simulink subsystem "Subsys_Conv_Electrical_Part_SPS"  (R2022b)
settings: Solver=VariableStepAuto  StartTime=0.0  StopTime=10.0  RelTol=1e-3
model mask{S_n=2e6, f_n=50, V_n_phph=690, V_n_grid_phph=20e3, T_s_ctrl=1e-3, T_s_meas=1e-4, T_s_SPS=1e-4, datatype='double', L_filter_conv_pu=[ 0.005 0.23 ], C_filter_pu=[ 0.005 0.01 ], L_filter_grid_pu=[ 0.01 0.04 ], withTransformer=1, RL_Trafo_Conv=[ 0.005 0.02 ], RL_Trafo_Grid=[ 0.005 0.02 ], Rm=500, Lm=500, inverterModel=1, R_snubber_pu=5e6, R_on_pu=1e-3, energySourceModel=1, C_dc_pu=0.75, K_p_DC=1.2, K_i_DC=2.4}
  mask prompts: S_n "Nominal Apparent Power [VA]"; f_n "Nominal Frequency [Hz]"; V_n_phph "Nominal Converter Voltage (rms, ph-ph) [V]"; V_n_grid_phph "Nominal Grid Voltage (rms, ph-ph) [V]"; T_s_ctrl "DC-link voltage controller sample time [s]"; T_s_meas "Measurement sample time [s]"; T_s_SPS "Simscape SPS sample time [s]"; datatype "Measurement signal data type"; L_filter_conv_pu "Impedance of Converter-Side-Inductor [ R L ] (p.u.)"; C_filter_pu "Impedance of Filter Capacitor [ R C ] (p.u.)"; L_filter_grid_pu "Impedance of Grid-Side-Inductor (only if no transformer used) [ R L ] (p.u.)"; withTransformer "Grid coupling: (1 = with transformer, 0 = direct grid coupling (without transformer)"; RL_Trafo_Conv "Converter-Side Impedance [ R L ] (pu):"; RL_Trafo_Grid "Grid-Side Impedance [ R L ] (pu):"; Rm "Magnetization resistance  Rm (pu):"; Lm "Magnetization inductance  Lm (pu):"; inverterModel "Modeling of inverter brigde: (1 = Average Model, 0 = Ideal Switches)"; R_snubber_pu "Snubber Resistance for Ideal Switches (pu)"; R_on_pu "On-State Resistance of Ideal Switches (pu)"; energySourceModel "Modeling of energy source (1 = power-limited DC current source , 0 = constant DC voltage)"; C_dc_pu "Capacitance of DC-link capacitor (pu)"; K_p_DC "Current controller proportional gain (pu)"; K_i_DC "Current controller integral gain (pu/s)"
undefined symbols (not defined in the file): D1, Delta
libraries: spsThreePhaseVIMeasurementLib x6, spsIdealSwitchLib x3, spsThreePhaseSeriesRLCBranchLib x3, spsUniversalBridgeLib x2, spsVoltageMeasurementLib x2, spsGroundLib x1, spsDCVoltageSourceLib x1, spsControlledCurrentSourceLib x1, slpidlib x1, spsSeriesRLCBranchLib x1, spsThreePhaseBreakerLib x1, spsThreePhaseTransformerTwoWindingsLib x1
settings Model: Creator=winkens  LastModifiedBy=winkens
settings SolverCC: AlgebraicLoopSolver=TrustRegion
settings DebuggingCC: UnconnectedInputMsg=warning  UnconnectedOutputMsg=warning  UnconnectedLineMsg=warning  SFMachineParentedDataDiag=warning
settings ModelReferenceCC: EnableRefExpFcnMdlSchedulingChecks=on
settings RTWCC: DLArmComputeVersion=19.05

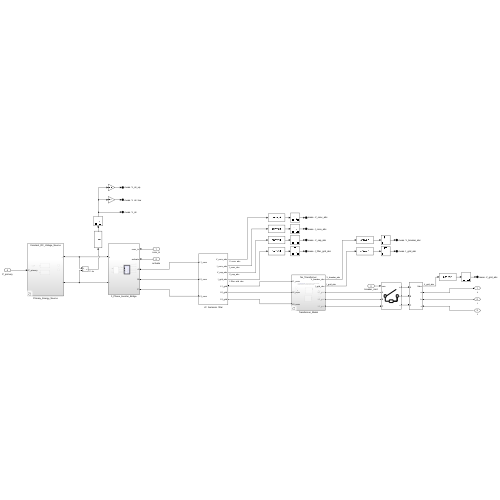
[thumbnail: Simulink's stored preview of the top-level diagram]
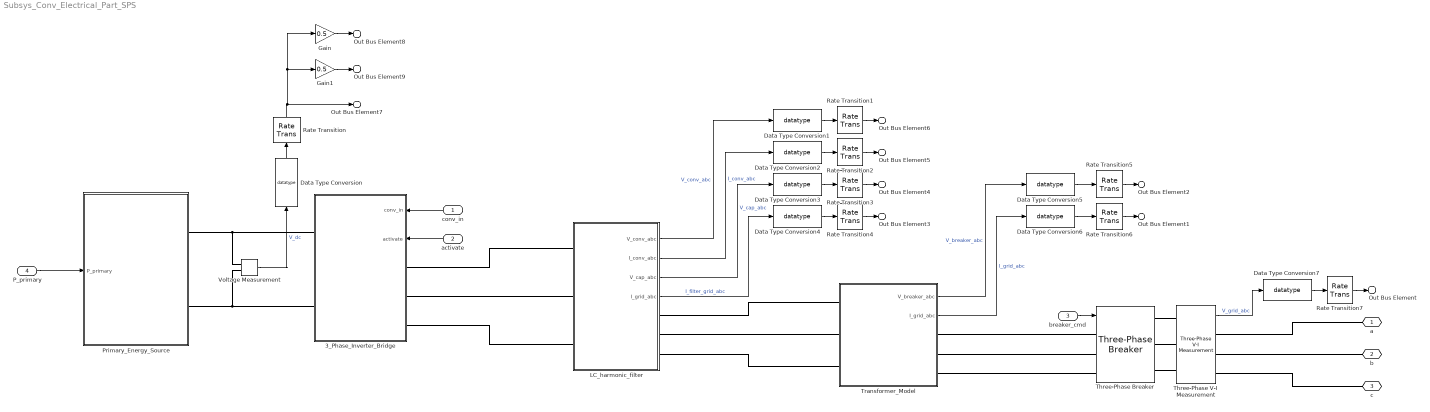
== system Subsys_Conv_Electrical_Part_SPS ==
  conv_in : Inport
  activate : Inport  Port=2
  breaker_cmd : Inport  Port=3
  P_primary : Inport  Port=4
  3_Phase_Inverter_Bridge : Subsystem
  Data Type Conversion{,1..7} (8 alike) : DataTypeConversion  OutDataTypeStr=datatype  SaturateOnIntegerOverflow=off  RndMeth=Floor
  Gain : Gain  Gain=0.5
  Gain1 : Gain  Gain=0.5
  LC_harmonic_filter : Subsystem
  Primary_Energy_Source : Subsystem  Variant=on
  Rate Transition{,1..7} (8 alike) : RateTransition  OutPortSampleTime=T_s_meas
  Three-Phase V-I Measurement : spsThreePhaseVIMeasurementLib/Three-Phase V-I Measurement  VoltageMeasurement=phase-to-ground  SetLabelV=off  LabelV=Vabc  Vpu=off  VpuLL=off  CurrentMeasurement=no  SetLabelI=off  LabelI=Iabc  Ipu=off  Pbase=100e6  Vbase=500e3  OutputType=Complex  PhasorSimulation=off  PSBequivalent=0
  Three-Phase Breaker : spsThreePhaseBreakerLib/Three-Phase Breaker  InitialState=open  SwitchA=on  SwitchB=on  SwitchC=on  SwitchTimes="[1/60  5/60]"  External=on  BreakerResistance=0.01  SnubberResistance=1e6  SnubberCapacitance=inf  Measurements=None
  Transformer_Model : Subsystem  Variant=on
  Voltage Measurement : spsVoltageMeasurementLib/Voltage Measurement  PhasorSimulation=off  OutputType=Complex  PSBequivalent=0
  a : PMIOPort  Side=Right
  b : PMIOPort  Port=2  Side=Right
  c : PMIOPort  Port=3  Side=Right
  Out Bus Element : Outport  PortName=meas  Element=V_grid_abc
  Out Bus Element1 : Outport  PortName=meas  Element=I_grid_abc
  Out Bus Element2 : Outport  PortName=meas  Element=V_breaker_abc
  Out Bus Element3 : Outport  PortName=meas  Element=I_filter_grid_abc
  Out Bus Element4 : Outport  PortName=meas  Element=V_cap_abc
  Out Bus Element5 : Outport  PortName=meas  Element=I_conv_abc
  Out Bus Element6 : Outport  PortName=meas  Element=V_conv_abc
  Out Bus Element7 : Outport  PortName=meas  Element=V_dc
  Out Bus Element8 : Outport  PortName=meas  Element=V_dc_up
  Out Bus Element9 : Outport  PortName=meas  Element=V_dc_low
  wires:
  LC_harmonic_filter/4(I_grid_abc) -> Data Type Conversion4/1  "I_filter_grid_abc"
  breaker_cmd/1 -> Three-Phase Breaker/1
  Transformer_Model/1(V_breaker_abc) -> Data Type Conversion5/1  "V_breaker_abc"
  LC_harmonic_filter/2(I_conv_abc) -> Data Type Conversion2/1  "I_conv_abc"
  LC_harmonic_filter/3(V_cap_abc) -> Data Type Conversion3/1  "V_cap_abc"
  Voltage Measurement/1 -> Data Type Conversion/1  "V_dc"
  Three-Phase V-I Measurement/1 -> Data Type Conversion7/1  "V_grid_abc"
  LC_harmonic_filter/1(V_conv_abc) -> Data Type Conversion1/1  "V_conv_abc"
  Transformer_Model/2(I_grid_abc) -> Data Type Conversion6/1  "I_grid_abc"
  P_primary/1 -> Primary_Energy_Source/1(P_primary)
  activate/1 -> 3_Phase_Inverter_Bridge/2(activate)
  conv_in/1 -> 3_Phase_Inverter_Bridge/1(conv_in)
  Gain/1 -> Out Bus Element8/1
  Gain1/1 -> Out Bus Element9/1
  Rate Transition/1 -> Out Bus Element7/1, Gain/1, Gain1/1
  Rate Transition1/1 -> Out Bus Element6/1
  Rate Transition2/1 -> Out Bus Element5/1
  Rate Transition3/1 -> Out Bus Element4/1
  Rate Transition4/1 -> Out Bus Element3/1
  Rate Transition5/1 -> Out Bus Element2/1
  Rate Transition6/1 -> Out Bus Element1/1
  Rate Transition7/1 -> Out Bus Element/1
  Data Type Conversion/1 -> Rate Transition/1
  Data Type Conversion1/1 -> Rate Transition1/1
  Data Type Conversion2/1 -> Rate Transition2/1
  Data Type Conversion3/1 -> Rate Transition3/1
  Data Type Conversion4/1 -> Rate Transition4/1
  Data Type Conversion5/1 -> Rate Transition5/1
  Data Type Conversion6/1 -> Rate Transition6/1
  Data Type Conversion7/1 -> Rate Transition7/1
  connections:
  Voltage Measurement/LConn1 -- Primary_Energy_Source/RConn1 -- 3_Phase_Inverter_Bridge/RConn1
  Primary_Energy_Source/RConn2 -- Voltage Measurement/LConn2 -- 3_Phase_Inverter_Bridge/RConn2
  Three-Phase V-I Measurement/RConn2 -- b/RConn1
  Three-Phase V-I Measurement/RConn1 -- a/RConn1
  LC_harmonic_filter/LConn3 -- 3_Phase_Inverter_Bridge/LConn3
  Three-Phase Breaker/LConn3 -- Transformer_Model/RConn3
  Three-Phase V-I Measurement/LConn2 -- Three-Phase Breaker/RConn2
  Three-Phase V-I Measurement/RConn3 -- c/RConn1
  Three-Phase V-I Measurement/LConn1 -- Three-Phase Breaker/RConn1
  Three-Phase V-I Measurement/LConn3 -- Three-Phase Breaker/RConn3
  Three-Phase Breaker/LConn1 -- Transformer_Model/RConn1
  LC_harmonic_filter/RConn1 -- Transformer_Model/LConn1
  Three-Phase Breaker/LConn2 -- Transformer_Model/RConn2
  LC_harmonic_filter/RConn3 -- Transformer_Model/LConn3
  Transformer_Model/LConn2 -- LC_harmonic_filter/RConn2
  LC_harmonic_filter/LConn1 -- 3_Phase_Inverter_Bridge/LConn1
  LC_harmonic_filter/LConn2 -- 3_Phase_Inverter_Bridge/LConn2

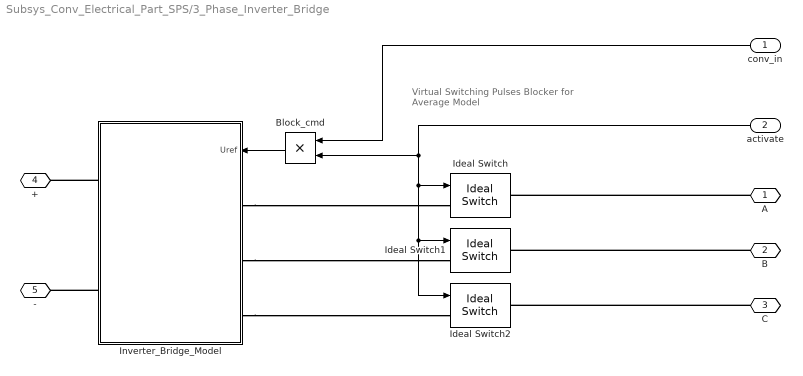
== system Subsys_Conv_Electrical_Part_SPS/3_Phase_Inverter_Bridge ==
  note: Virtual Switching Pulses
      | Blocker for Average Model
  conv_in : Inport
  activate : Inport  Port=2
  Block_cmd : Product  Inputs=**
  Ideal Switch : spsIdealSwitchLib/Ideal Switch  Ron=1e-6 * V_n_phph * V_n_phph / S_n  Lon=0  IC=1  Rs=1e6 * V_n_phph * V_n_phph / S_n  Cs=inf  Measurements=off
  Ideal Switch1 : spsIdealSwitchLib/Ideal Switch  Ron=1e-6 * V_n_phph * V_n_phph / S_n  Lon=0  IC=1  Rs=1e6 * V_n_phph * V_n_phph / S_n  Cs=inf  Measurements=off
  Ideal Switch2 : spsIdealSwitchLib/Ideal Switch  Ron=1e-6 * V_n_phph * V_n_phph / S_n  Lon=0  IC=1  Rs=1e6 * V_n_phph * V_n_phph / S_n  Cs=inf  Measurements=off
  Inverter_Bridge_Model : Subsystem  Variant=on  VariantControl=Choice
  A : PMIOPort  Side=Left
  B : PMIOPort  Port=2  Side=Left
  C : PMIOPort  Port=3  Side=Left
  + : PMIOPort  Port=4  Side=Right
  - : PMIOPort  Port=5  Side=Right
  wires:
  conv_in/1 -> Block_cmd/1
  activate/1 -> Ideal Switch/1, Ideal Switch1/1, Ideal Switch2/1, Block_cmd/2
  Block_cmd/1 -> Inverter_Bridge_Model/1(Uref)
  connections:
  C/RConn1 -- Ideal Switch2/RConn1
  B/RConn1 -- Ideal Switch1/RConn1
  A/RConn1 -- Ideal Switch/RConn1
  Inverter_Bridge_Model/LConn1 -- Ideal Switch/LConn1
  Inverter_Bridge_Model/LConn2 -- Ideal Switch1/LConn1
  Inverter_Bridge_Model/LConn3 -- Ideal Switch2/LConn1
  Inverter_Bridge_Model/RConn1 -- +/RConn1
  Inverter_Bridge_Model/RConn2 -- -/RConn1

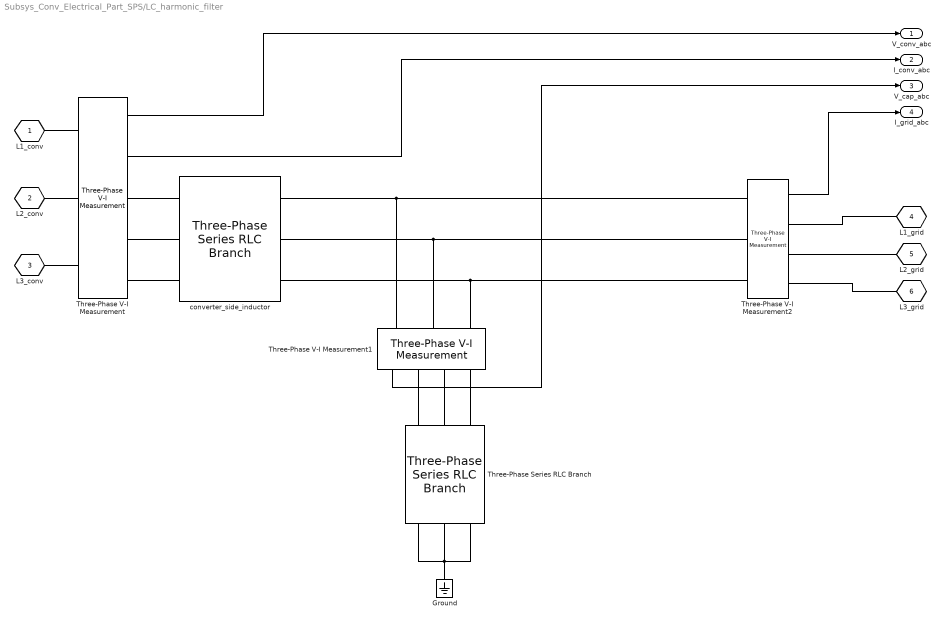
== system Subsys_Conv_Electrical_Part_SPS/LC_harmonic_filter ==
  Ground : spsGroundLib/Ground  LConnTagsString=a
  Three-Phase Series RLC Branch : spsThreePhaseSeriesRLCBranchLib/Three-Phase Series RLC Branch  LConnTagsString=A|B|C  RConnTagsString=A|B|C  BranchType=RC  Resistance=C_filter_pu(1)*V_n_phph*V_n_phph/S_n  Inductance=1e-3  Capacitance=C_filter_pu(2)*S_n/(2*pi*50*V_n_phph*V_n_phph)  Measurements=None
  Three-Phase V-I Measurement : spsThreePhaseVIMeasurementLib/Three-Phase V-I Measurement  VoltageMeasurement=phase-to-ground  SetLabelV=off  LabelV=Vabc  Vpu=off  VpuLL=off  CurrentMeasurement=yes  SetLabelI=off  LabelI=Iabc  Ipu=off  Pbase=100e6  Vbase=500e3  OutputType=Complex  PhasorSimulation=off  PSBequivalent=0
  Three-Phase V-I Measurement1 : spsThreePhaseVIMeasurementLib/Three-Phase V-I Measurement  VoltageMeasurement=phase-to-ground  SetLabelV=off  LabelV=Vabc  Vpu=off  VpuLL=off  CurrentMeasurement=no  SetLabelI=off  LabelI=Iabc  Ipu=off  Pbase=100e6  Vbase=500e3  OutputType=Complex  PhasorSimulation=off  PSBequivalent=0
  Three-Phase V-I Measurement2 : spsThreePhaseVIMeasurementLib/Three-Phase V-I Measurement  VoltageMeasurement=no  SetLabelV=off  LabelV=Vabc  Vpu=off  VpuLL=off  CurrentMeasurement=yes  SetLabelI=off  LabelI=Iabc  Ipu=off  Pbase=100e6  Vbase=500e3  OutputType=Complex  PhasorSimulation=off  PSBequivalent=0
  converter_side_inductor : spsThreePhaseSeriesRLCBranchLib/Three-Phase Series RLC Branch  LConnTagsString=A|B|C  RConnTagsString=A|B|C  BranchType=RL  Resistance=L_filter_conv_pu(1)*V_n_phph*V_n_phph/S_n  Inductance=L_filter_conv_pu(2)*V_n_phph*V_n_phph/(2*pi*f_n*S_n)  Capacitance=1e-6  Measurements=None
  L1_conv : PMIOPort  Tag=PMCPort  Side=Left
  L2_conv : PMIOPort  Tag=PMCPort  Port=2  Side=Left
  L3_conv : PMIOPort  Tag=PMCPort  Port=3  Side=Left
  L1_grid : PMIOPort  Tag=PMCPort  Port=4  Side=Right
  L2_grid : PMIOPort  Tag=PMCPort  Port=5  Side=Right
  L3_grid : PMIOPort  Tag=PMCPort  Port=6  Side=Right
  V_conv_abc : Outport
  I_conv_abc : Outport  Port=2
  V_cap_abc : Outport  Port=3
  I_grid_abc : Outport  Port=4
  wires:
  Three-Phase V-I Measurement/1 -> V_conv_abc/1
  Three-Phase V-I Measurement1/1 -> V_cap_abc/1
  Three-Phase V-I Measurement2/1 -> I_grid_abc/1
  Three-Phase V-I Measurement/2 -> I_conv_abc/1
  connections:
  Three-Phase V-I Measurement1/LConn3 -- Three-Phase V-I Measurement2/LConn3 -- converter_side_inductor/RConn3
  Three-Phase V-I Measurement1/LConn1 -- Three-Phase V-I Measurement2/LConn1 -- converter_side_inductor/RConn1
  Three-Phase V-I Measurement2/RConn3 -- L3_grid/RConn1
  Three-Phase V-I Measurement2/RConn2 -- L2_grid/RConn1
  Three-Phase V-I Measurement2/RConn1 -- L1_grid/RConn1
  Three-Phase V-I Measurement1/LConn2 -- Three-Phase V-I Measurement2/LConn2 -- converter_side_inductor/RConn2
  Three-Phase Series RLC Branch/LConn3 -- Three-Phase V-I Measurement1/RConn3
  Three-Phase Series RLC Branch/LConn2 -- Three-Phase V-I Measurement1/RConn2
  Three-Phase Series RLC Branch/LConn1 -- Three-Phase V-I Measurement1/RConn1
  Three-Phase Series RLC Branch/RConn2 -- Three-Phase Series RLC Branch/RConn1 -- Three-Phase Series RLC Branch/RConn3 -- Ground/LConn1
  Three-Phase V-I Measurement/RConn3 -- converter_side_inductor/LConn3
  Three-Phase V-I Measurement/RConn2 -- converter_side_inductor/LConn2
  Three-Phase V-I Measurement/RConn1 -- converter_side_inductor/LConn1
  Three-Phase V-I Measurement/LConn3 -- L3_conv/RConn1
  Three-Phase V-I Measurement/LConn2 -- L2_conv/RConn1
  Three-Phase V-I Measurement/LConn1 -- L1_conv/RConn1

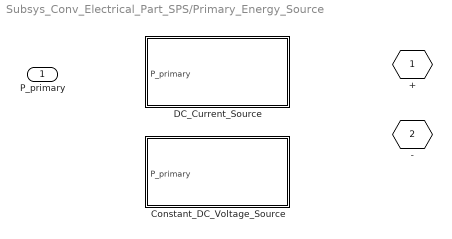
== system Subsys_Conv_Electrical_Part_SPS/Primary_Energy_Source ==
  P_primary : Inport
  Constant_DC_Voltage_Source : Subsystem  VariantControl=energySourceModel == 0
  DC_Current_Source : Subsystem  VariantControl=(default)
  + : PMIOPort  Tag=PMCPort  Side=Right
  - : PMIOPort  Tag=PMCPort  Port=2  Side=Right

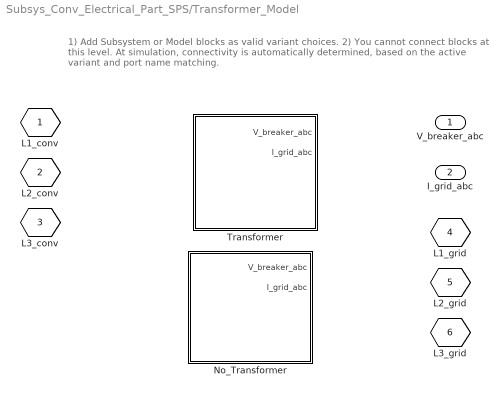
== system Subsys_Conv_Electrical_Part_SPS/Transformer_Model ==
  note: 1) Add Subsystem or Model blocks as valid variant choices.
      | 2) You cannot connect blocks at this level. At simulation, connectivity is automatically
      | determined, based on the active variant and port name matching.
  No_Transformer : Subsystem  VariantControl=withTransformer == 0
  Transformer : Subsystem  VariantControl=(default)
  L1_conv : PMIOPort  Tag=PMCPort  Side=Left
  L2_conv : PMIOPort  Tag=PMCPort  Port=2  Side=Left
  L3_conv : PMIOPort  Tag=PMCPort  Port=3  Side=Left
  L1_grid : PMIOPort  Tag=PMCPort  Port=4  Side=Right
  L2_grid : PMIOPort  Tag=PMCPort  Port=5  Side=Right
  L3_grid : PMIOPort  Tag=PMCPort  Port=6  Side=Right
  V_breaker_abc : Outport
  I_grid_abc : Outport  Port=2

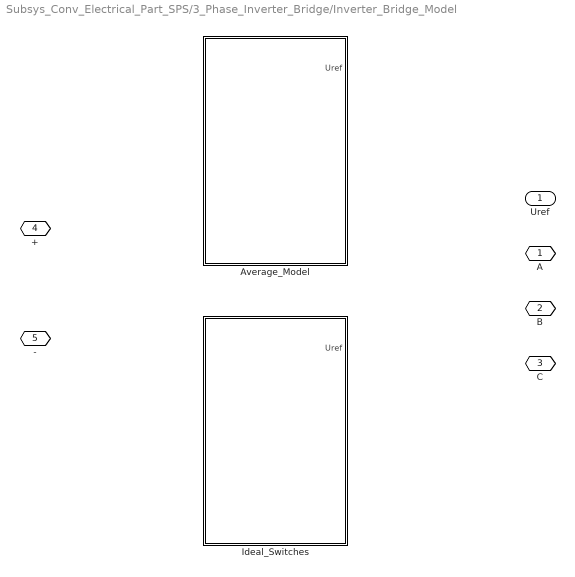
== system Subsys_Conv_Electrical_Part_SPS/3_Phase_Inverter_Bridge/Inverter_Bridge_Model ==
  Uref : Inport
  Average_Model : Subsystem  VariantControl=(default)
  Ideal_Switches : Subsystem  VariantControl=inverterModel == 0
  A : PMIOPort  Side=Left
  B : PMIOPort  Port=2  Side=Left
  C : PMIOPort  Port=3  Side=Left
  + : PMIOPort  Port=4  Side=Right
  - : PMIOPort  Port=5  Side=Right

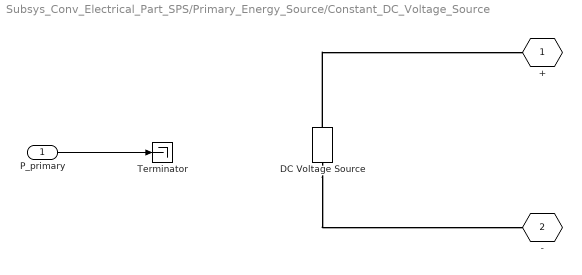
== system Subsys_Conv_Electrical_Part_SPS/Primary_Energy_Source/Constant_DC_Voltage_Source ==
  P_primary : Inport
  DC Voltage Source : spsDCVoltageSourceLib/DC Voltage Source  Amplitude=2*V_n_phph  Measurements=None
  Terminator : Terminator
  + : PMIOPort  Tag=PMCPort  Side=Right
  - : PMIOPort  Tag=PMCPort  Port=2  Side=Right
  wires:
  P_primary/1 -> Terminator/1
  connections:
  DC Voltage Source/LConn1 -- -/RConn1
  DC Voltage Source/RConn1 -- +/RConn1

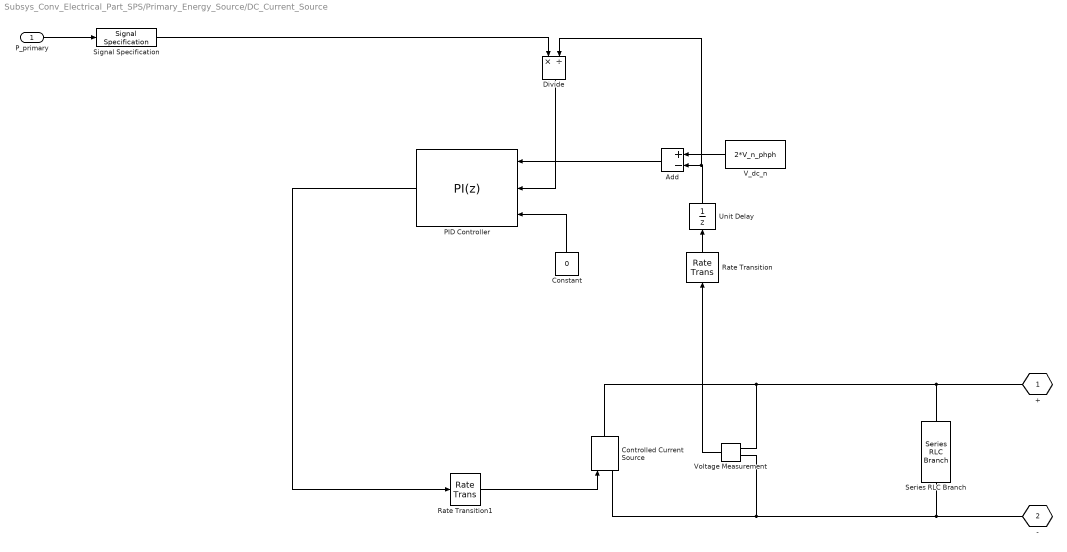
== system Subsys_Conv_Electrical_Part_SPS/Primary_Energy_Source/DC_Current_Source ==
  P_primary : Inport
  Add : Sum  Inputs=+-
  Constant : Constant  Value=0
  Controlled Current Source : spsControlledCurrentSourceLib/Controlled Current Source  Initialize=on  Source_Type=DC  Amplitude=0  Phase=0  Frequency=0  Measurements=None
  Divide : Product  Inputs=*/
  PID Controller : slpidlib/PID Controller  Controller=PI  Form=Parallel  TimeDomain=Discrete-time  UseExternalTs=off  SampleTime=T_s_ctrl  IntegratorMethod=Forward Euler  FilterMethod=Forward Euler  ControllerParametersSource=internal  P=K_p_DC*S_n/(V_n_phph*V_n_phph)  I=K_i_DC*S_n/(V_n_phph*V_n_phph)  D=0  UseFilter=on  N=100  TunerSelectOption=Transfer Function Based (PID Tuner App)  InitialConditionSource=internal  InitialConditionForIntegrator=0  InitialConditionForFilter=0  DifferentiatorICPrevScaledInput=0  ExternalReset=none  TrackingMode=off  Kt=1  LimitOutput=on  SatLimitsSource=external  UpperSaturationLimit=inf  LowerSaturationLimit=-inf  LinearizeAsGain=on  AntiWindupMode=clamping  Kb=1  POutMin=[]  POutMax=[]  IOutMin=[]  IOutMax=[]  DOutMin=[]  DOutMax=[]  NOutMin=[]  NOutMax=[]  SumOutMin=[]  SumOutMax=[]  SaturationOutMin=[]  SaturationOutMax=[]  PParamMin=[]  PParamMax=[]  IParamMin=[]  IParamMax=[]  DParamMin=[]  DParamMax=[]  NParamMin=[]  NParamMax=[]  KbParamMin=[]  KbParamMax=[]  KtParamMin=[]  KtParamMax=[]  KbOutMin=[]  KbOutMax=[]  KtOutMin=[]  KtOutMax=[]  IntegratorOutMin=[]  IntegratorOutMax=[]  FilterOutMin=[]  FilterOutMax=[]  SumI1OutMin=[]  SumI1OutMax=[]  SumI2OutMin=[]  SumI2OutMax=[]  SumI3OutMin=[]  SumI3OutMax=[]  SumI4OutMin=[]  SumI4OutMax=[]  SumDOutMin=[]  SumDOutMax=[]  DifferentiatorOutMin=[]  DifferentiatorOutMax=[]  FilterDiffOutCoefMin=[]  FilterDiffOutCoefMax=[]  ReciprocalOutMin=[]  ReciprocalOutMax=[]  SumDenOutMin=[]  SumDenOutMax=[]  SumNumOutMin=[]  SumNumOutMax=[]  DivideOutMin=[]  DivideOutMax=[]  UdiffTsProdOutMin=[]  UdiffTsProdOutMax=[]  NTsProdOutMin=[]  NTsProdOutMax=[]  UintegralTsProdOutMin=[]  UintegralTsProdOutMax=[]  UngainTsProdOutMin=[]  UngainTsProdOutMax=[]  IntegratorContinuousStateAttributes=''  IntegratorStateMustResolveToSignalObject=off  IntegratorRTWStateStorageClass=Auto  FilterContinuousStateAttributes=''  FilterStateMustResolveToSignalObject=off  FilterRTWStateStorageClass=Auto  ParallelPVariant=InternalParameters  IdealPVariant=Disabled  IVariant=InternalParameters  DVariant=Disabled  IntegratorVariant=Discrete  SatVariant=External  AWVariant=DiscClampingParallel  PCopyVariant=Disabled  TRVariant=Disabled  FdbkBlocksVariant=Forward  IdealPFdbkVariant=Disabled  SatFdbkVariant=Disabled  DerivativeFilterVariant=Disabled  NVariant=Disabled  NCopyVariant=Disabled_SignalSpec  FilterICVariant=Disabled  IntegratorICVariant=InternalICs  ExternalResetVariant=Disabled  TRSumVariant=Passthrough  SumFdbkVariant=Disabled  SumVariant=Sum_PI  TsampFilterVariant=InternalTs  TsampNgainVariant=Passthrough  TsampIntegralVariant=Passthrough  ExternalSaturationOutDataTypeStr=Inherit: Same as second input
  Rate Transition : RateTransition  OutPortSampleTime=T_s_ctrl
  Rate Transition1 : RateTransition  Deterministic=off  OutPortSampleTime=T_s_SPS
  Series RLC Branch : spsSeriesRLCBranchLib/Series RLC Branch  LConnTagsString=__new0  RConnTagsString=__new0  BranchType=C  Resistance=1  Inductance=1e-3  SetiL0=off  InitialCurrent=0  Capacitance=C_dc_pu*S_n/(2*pi*f_n*V_n_phph*V_n_phph)  Setx0=on  InitialVoltage=2*V_n_phph  Measurements=None
  Signal Specification : SignalSpecification  SampleTime=T_s_ctrl
  Unit Delay : UnitDelay  InitialCondition=2*V_n_phph  SampleTime=-1  HasFrameUpgradeWarning=on
  V_dc_n : Constant  Value=2*V_n_phph
  Voltage Measurement : spsVoltageMeasurementLib/Voltage Measurement  PhasorSimulation=off  OutputType=Complex  PSBequivalent=0
  + : PMIOPort  Tag=PMCPort  Side=Right
  - : PMIOPort  Tag=PMCPort  Port=2  Side=Right
  wires:
  PID Controller/1 -> Rate Transition1/1
  P_primary/1 -> Signal Specification/1
  Add/1 -> PID Controller/1
  V_dc_n/1 -> Add/1
  Unit Delay/1 -> Add/2, Divide/2
  Constant/1 -> PID Controller/3
  Divide/1 -> PID Controller/2
  Rate Transition/1 -> Unit Delay/1
  Signal Specification/1 -> Divide/1
  Voltage Measurement/1 -> Rate Transition/1
  Rate Transition1/1 -> Controlled Current Source/1
  connections:
  Controlled Current Source/LConn1 -- Voltage Measurement/LConn2 -- -/RConn1 -- Series RLC Branch/RConn1
  Controlled Current Source/RConn1 -- Voltage Measurement/LConn1 -- +/RConn1 -- Series RLC Branch/LConn1

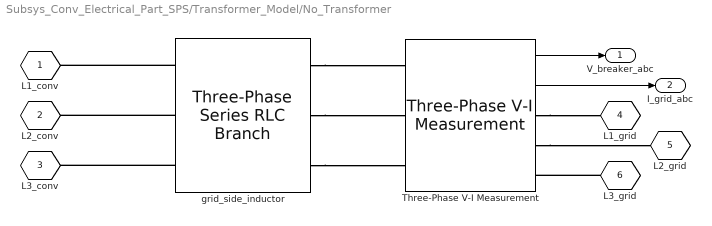
== system Subsys_Conv_Electrical_Part_SPS/Transformer_Model/No_Transformer ==
  Three-Phase V-I Measurement : spsThreePhaseVIMeasurementLib/Three-Phase V-I Measurement  VoltageMeasurement=phase-to-ground  SetLabelV=off  LabelV=Vabc  Vpu=off  VpuLL=off  CurrentMeasurement=yes  SetLabelI=off  LabelI=Iabc  Ipu=off  Pbase=100e6  Vbase=500e3  OutputType=Complex  PhasorSimulation=off  PSBequivalent=0
  grid_side_inductor : spsThreePhaseSeriesRLCBranchLib/Three-Phase Series RLC Branch  LConnTagsString=A|B|C  RConnTagsString=A|B|C  BranchType=RL  Resistance=L_filter_grid_pu(1)*V_n_phph*V_n_phph/S_n  Inductance=L_filter_grid_pu(2)*V_n_phph*V_n_phph/(2*pi*f_n*S_n)  Capacitance=1e-6  Measurements=None
  L1_conv : PMIOPort  Tag=PMCPort  Side=Left
  L2_conv : PMIOPort  Tag=PMCPort  Port=2  Side=Left
  L3_conv : PMIOPort  Tag=PMCPort  Port=3  Side=Left
  L1_grid : PMIOPort  Tag=PMCPort  Port=4  Side=Right
  L2_grid : PMIOPort  Tag=PMCPort  Port=5  Side=Right
  L3_grid : PMIOPort  Tag=PMCPort  Port=6  Side=Right
  V_breaker_abc : Outport
  I_grid_abc : Outport  Port=2
  wires:
  Three-Phase V-I Measurement/1 -> V_breaker_abc/1
  Three-Phase V-I Measurement/2 -> I_grid_abc/1
  connections:
  grid_side_inductor/LConn3 -- L3_conv/RConn1
  grid_side_inductor/LConn2 -- L2_conv/RConn1
  grid_side_inductor/LConn1 -- L1_conv/RConn1
  grid_side_inductor/RConn1 -- Three-Phase V-I Measurement/LConn1
  grid_side_inductor/RConn2 -- Three-Phase V-I Measurement/LConn2
  grid_side_inductor/RConn3 -- Three-Phase V-I Measurement/LConn3
  Three-Phase V-I Measurement/RConn1 -- L1_grid/RConn1
  Three-Phase V-I Measurement/RConn2 -- L2_grid/RConn1
  L3_grid/RConn1 -- Three-Phase V-I Measurement/RConn3

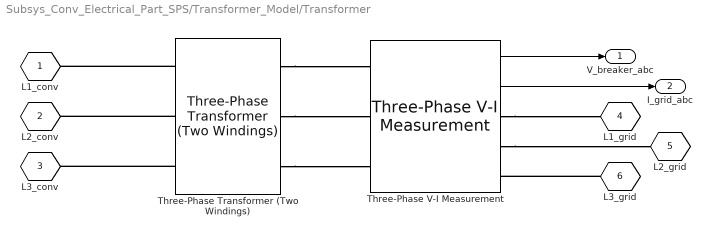
== system Subsys_Conv_Electrical_Part_SPS/Transformer_Model/Transformer ==
  Three-Phase Transformer (Two Windings) : spsThreePhaseTransformerTwoWindingsLib/Three-Phase Transformer (Two Windings)  Winding1Connection=Yg  Winding2Connection=Delta (D1)  CoreType=Three-limb core (core-type)  SetSaturation=off  Hysteresis=off  DataFile='hysteresis'  SetInitialFlux=off  Measurements=None  UNITS=pu  NominalPower=[ S_n , f_n ]  Winding1=[ V_n_phph , RL_Trafo_Conv(1) , RL_Trafo_Conv(2) ]  Winding2=[ 1.02*V_n_grid_phph , RL_Trafo_Grid(1) , RL_Trafo_Grid(2) ]  Rm=Rm  Lm=Lm  L0=0.5  Saturation=[ 0,0 ; 0.0024,1.2 ; 1.0,1.52 ]  InitialFluxes=[ 0.8 , -0.8 , 0.7 ]  BreakLoop=off  DiscreteSolver=Trapezoidal iterative  DataType=off  TransfoNumber=1
  Three-Phase V-I Measurement : spsThreePhaseVIMeasurementLib/Three-Phase V-I Measurement  VoltageMeasurement=phase-to-ground  SetLabelV=off  LabelV=Vabc  Vpu=off  VpuLL=off  CurrentMeasurement=yes  SetLabelI=off  LabelI=Iabc  Ipu=off  Pbase=100e6  Vbase=500e3  OutputType=Complex  PhasorSimulation=off  PSBequivalent=0
  L1_conv : PMIOPort  Tag=PMCPort  Side=Left
  L2_conv : PMIOPort  Tag=PMCPort  Port=2  Side=Left
  L3_conv : PMIOPort  Tag=PMCPort  Port=3  Side=Left
  L1_grid : PMIOPort  Tag=PMCPort  Port=4  Side=Right
  L2_grid : PMIOPort  Tag=PMCPort  Port=5  Side=Right
  L3_grid : PMIOPort  Tag=PMCPort  Port=6  Side=Right
  V_breaker_abc : Outport
  I_grid_abc : Outport  Port=2
  wires:
  Three-Phase V-I Measurement/1 -> V_breaker_abc/1
  Three-Phase V-I Measurement/2 -> I_grid_abc/1
  connections:
  Three-Phase Transformer (Two Windings)/LConn3 -- L3_conv/RConn1
  Three-Phase Transformer (Two Windings)/LConn2 -- L2_conv/RConn1
  Three-Phase Transformer (Two Windings)/LConn1 -- L1_conv/RConn1
  Three-Phase Transformer (Two Windings)/RConn3 -- Three-Phase V-I Measurement/LConn3
  Three-Phase Transformer (Two Windings)/RConn2 -- Three-Phase V-I Measurement/LConn2
  Three-Phase Transformer (Two Windings)/RConn1 -- Three-Phase V-I Measurement/LConn1
  Three-Phase V-I Measurement/RConn1 -- L1_grid/RConn1
  Three-Phase V-I Measurement/RConn2 -- L2_grid/RConn1
  L3_grid/RConn1 -- Three-Phase V-I Measurement/RConn3

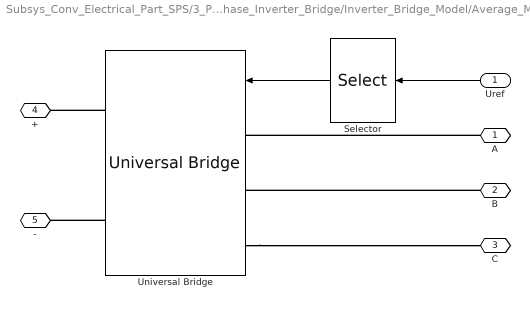
== system Subsys_Conv_Electrical_Part_SPS/3_Phase_Inverter_Bridge/Inverter_Bridge_Model/Average_Model ==
  Uref : Inport
  Selector : Selector  InputPortWidth=6  IndexOptions=Index vector (dialog)  Indices=[1 2 3]  OutputSizes=1
  Universal Bridge : spsUniversalBridgeLib/Universal Bridge  Arms=3  SnubberResistance=1e6  SnubberCapacitance=inf  Device=Average-model based VSC  Ron=1e-3  Lon=0  ForwardVoltages="[  0  0  ]"  ForwardVoltage=0  GTOparameters=[ 10e-6 , 20e-6 ]  IGBTparameters=[ 1e-6 , 2e-6 ]  Measurements=None  Measurements_2=None  converterType=Rectifier
  A : PMIOPort  Side=Left
  B : PMIOPort  Port=2  Side=Left
  C : PMIOPort  Port=3  Side=Left
  + : PMIOPort  Port=4  Side=Right
  - : PMIOPort  Port=5  Side=Right
  wires:
  Uref/1 -> Selector/1
  Selector/1 -> Universal Bridge/1
  connections:
  Universal Bridge/LConn3 -- C/RConn1
  B/RConn1 -- Universal Bridge/LConn2
  Universal Bridge/RConn2 -- -/RConn1
  Universal Bridge/RConn1 -- +/RConn1
  A/RConn1 -- Universal Bridge/LConn1

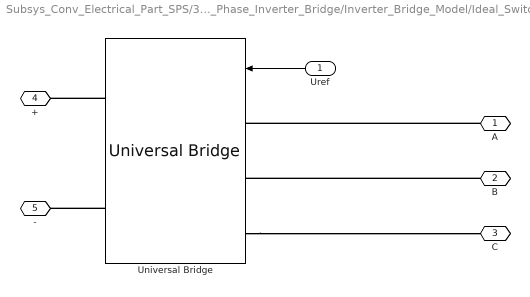
== system Subsys_Conv_Electrical_Part_SPS/3_Phase_Inverter_Bridge/Inverter_Bridge_Model/Ideal_Switches ==
  Uref : Inport
  Universal Bridge : spsUniversalBridgeLib/Universal Bridge  Arms=3  SnubberResistance=R_snubber_pu*V_n_phph*V_n_phph/S_n  SnubberCapacitance=inf  Device=Ideal Switches  Ron=R_on_pu*V_n_phph*V_n_phph/S_n  Lon=0  ForwardVoltages="[  0  0  ]"  ForwardVoltage=0  GTOparameters=[ 10e-6 , 20e-6 ]  IGBTparameters=[ 1e-6 , 2e-6 ]  Measurements=None  Measurements_2=None  converterType=Rectifier
  A : PMIOPort  Side=Left
  B : PMIOPort  Port=2  Side=Left
  C : PMIOPort  Port=3  Side=Left
  + : PMIOPort  Port=4  Side=Right
  - : PMIOPort  Port=5  Side=Right
  wires:
  Uref/1 -> Universal Bridge/1
  connections:
  Universal Bridge/LConn3 -- C/RConn1
  B/RConn1 -- Universal Bridge/LConn2
  Universal Bridge/RConn2 -- -/RConn1
  Universal Bridge/RConn1 -- +/RConn1
  A/RConn1 -- Universal Bridge/LConn1
